simulink model "chaine_gauss"  (R2023b)
settings: Solver=FixedStepDiscrete  StartTime=0.0  StopTime=10.0  FixedStep=Tb/L  RelTol=1e-3
values from neighbouring files (symbols this model uses):
  A = P.A    [Parametres.m]
  graine = round(P.graine)    [Parametres.m]    (also in parametres_perso.m = mod(sum(c .* (1:numel(c)) * 31) + 7 * numel(c), 2^31 - 1))
  L = P.L    [Parametres.m]
  seuil = 0    [Parametres.m]
  sigma2 = N0 * L / (2*Tb)    [Parametres.m]    (also in partie3.m; partie3_q12.m; partie4.m = N0 * L / (2 * Tb))
  Tb = 1    [Parametres.m]
settings Model: Creator=e2508348  LastModifiedBy=e2508348

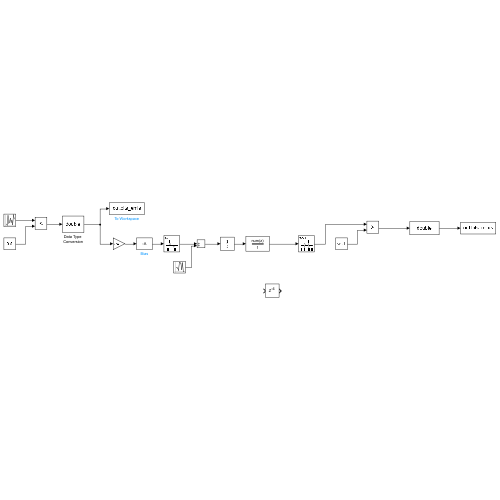
[thumbnail: Simulink's stored preview of the top-level diagram]
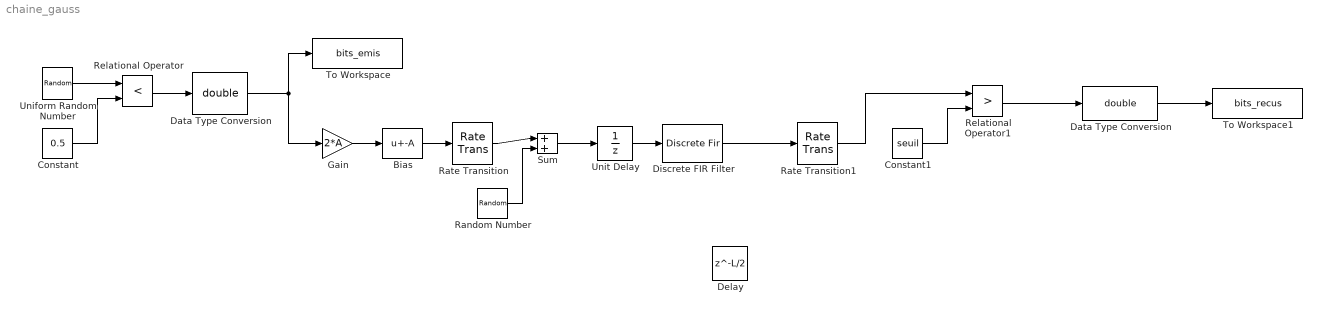
== system chaine_gauss ==
  Bias : Bias  Bias=-A  SaturateOnIntegerOverflow=off
  Constant : Constant  Value=0.5
  Constant1 : Constant  Value=seuil
  Data Type Conversion : DataTypeConversion  OutDataTypeStr=double  SaturateOnIntegerOverflow=off  RndMeth=Floor
  Data Type Conversion : DataTypeConversion  OutDataTypeStr=double  SaturateOnIntegerOverflow=off  RndMeth=Floor
  Delay : Delay  DelayLength=L/2
  Discrete FIR Filter : DiscreteFir  Coefficients=ones(1,L)/L
  Gain : Gain  Gain=2*A
  Random Number : RandomNumber  Variance=sigma2  Seed=graine+2  SampleTime=Tb/L
  Rate Transition : RateTransition  OutPortSampleTime=Tb/L
  Rate Transition1 : RateTransition  OutPortSampleTime=Tb
  Relational Operator : RelationalOperator  Operator=<  OutDataTypeStr=boolean  RndMeth=Simplest  InputSameDT=off
  Relational Operator1 : RelationalOperator  Operator=>  OutDataTypeStr=boolean  RndMeth=Simplest  InputSameDT=off
  Sum : Sum  Inputs=|++
  To Workspace : ToWorkspace  VariableName=bits_emis  SampleTime=-1
  To Workspace1 : ToWorkspace  VariableName=bits_recus  SampleTime=-1
  Uniform Random Number : UniformRandomNumber  Minimum=0  Seed=graine  SampleTime=Tb
  Unit Delay : UnitDelay  SampleTime=-1  HasFrameUpgradeWarning=on
  wires:
  Uniform Random Number/1 -> Relational Operator/1
  Constant/1 -> Relational Operator/2
  Relational Operator/1 -> Data Type Conversion/1
  Data Type Conversion/1 -> Gain/1, To Workspace/1
  Gain/1 -> Bias/1
  Bias/1 -> Rate Transition/1
  Rate Transition/1 -> Sum/1
  Random Number/1 -> Sum/2
  Sum/1 -> Unit Delay/1
  Unit Delay/1 -> Discrete FIR Filter/1
  Discrete FIR Filter/1 -> Rate Transition1/1
  Rate Transition1/1 -> Relational Operator1/1
  Constant1/1 -> Relational Operator1/2
  Relational Operator1/1 -> Data Type Conversion/1
  Data Type Conversion/1 -> To Workspace1/1
